simulink model "Disha_plant"  (R2026a)
settings: Solver=VariableStepAuto
settings Model: Creator=LENOVO  LastModifiedBy=LENOVO

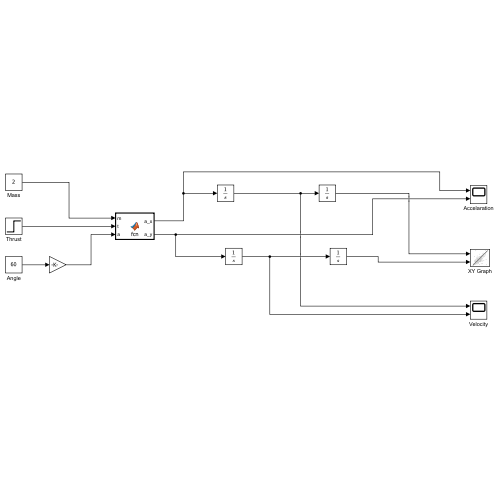
[thumbnail: Simulink's stored preview of the top-level diagram]
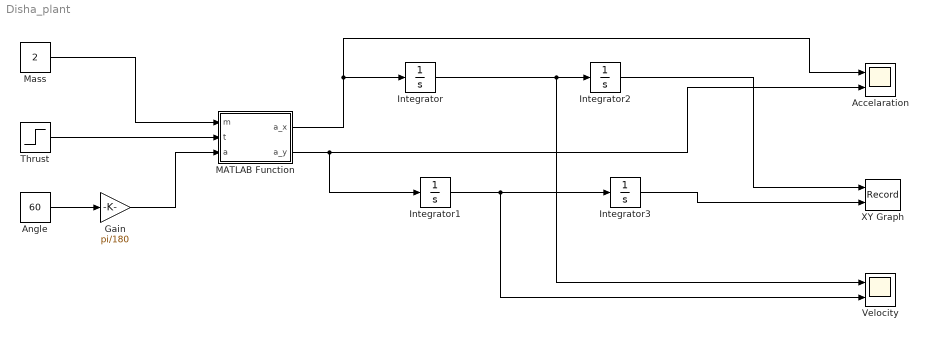
== system Disha_plant ==
  Accelaration : Scope  NumInputPorts=2
      settings: ActiveDisplayYMinimum=-0.0541265877365274  ActiveDisplayYMaximum=0.4871392896287467
  Angle : Constant  Value=60
  Gain : Gain  Gain=pi/180
  Integrator{,1..3} (4 alike) : Integrator
  MATLAB Function : MATLAB Function  TreatAsAtomicUnit=on
  Mass : Constant  Value=2
  Thrust : Step  SampleTime=0
  Velocity : Scope  NumInputPorts=2
      settings: ActiveDisplayYMinimum=-0.48713928962874653  ActiveDisplayYMaximum=4.38425360665872  DataLoggingVariableName=ScopeData2
  XY Graph : Record  NumPorts=2.0  FileSettingsInternal="{\"entries\":[{\"content\":{\"excelSettings\":{\"content\":{},\"type\":\"Streamout.ExcelSettings\"},\"parquetSettings\":{\"content\":{},\"type\":\"Streamout.ParquetSettings\"}},\"type\":\"Streamout.FileSettingStorage\",\"uuid\":\"\"}],\"packageUris\":[\"http:\\/\\/schema.mathworks.com\\/mf0\\/streamout_blocks\\/R2020a\"],\"version\":\"1.0\"}"  FrameSettings=[0, 0]  Layout=[1 1]  SignalsInternal="{\"entries\":[{\"content\":{\"signals\":[{\"content\":{\"blockPath\":[],\"dimensions\":[1],\"domain\":\"\",\"lineColor\":\"#a2142f\",\"plots\":[ 1 ],\"port\":1,\"sid\":[\"\"],\"signalID\":1,\"signalName\":\"Integrator2\"},\"type\":\"RecordBlkView.Signal\",\"uuid\":\"\"},{\"content\":{\"blockPath\":[],\"dimensions\":[1],\"domain\":\"\",\"lineColor\":\"#139fff\",\"plots\":[ 1 ],\"port\":2,\"sid\":[\"\"],\"signalID\":2,\"signalName\":\"Integrator3\"},\"type\":\"RecordBlkView.Signal\",\"uuid\":\"\"}]},\"type\":\"RecordBlkView.InputSignals\",\"uuid\":\"\"}],\"packageUris\":[\"http:\\/\\/schema.mathworks.com\\/mf0\\/streamout_blocks\\/R2020a\"],\"version\":\"1.0\"}"  VisualizationBindings="{\"xyplotplugin\":{\"info\":[{\"series\":[{\"bindingParametersList\":[{\"parameter\":\"X-Axis\",\"signalID\":1,\"signalName\":\"Integrator2\"},{\"parameter\":\"Y-Axis\",\"signalID\":2,\"signalName\":\"Integrator3\"}],\"seriesID\":0}],\"subplotID\":1}]}}"  CompatibilityTag=XY
  wires:
  Mass/1 -> MATLAB Function/1(m)
  Thrust/1 -> MATLAB Function/2(t)
  Angle/1 -> Gain/1
  Gain/1 -> MATLAB Function/3(a)
  MATLAB Function/2(a_y) -> Accelaration/2, Integrator1/1
  Integrator1/1 -> Velocity/2, Integrator3/1
  Integrator2/1 -> XY Graph/1
  Integrator3/1 -> XY Graph/2
  MATLAB Function/1(a_x) -> Accelaration/1, Integrator/1
  Integrator/1 -> Velocity/1, Integrator2/1

== matlab function Disha_plant/MATLAB Function ==
  data: m input; a_x output; t input; a input; a_y output
function [a_x, a_y] = fcn(m, t, a)
% Inputs:
%   m - mass (kg)
%   t - thrust (N)
%   a - thrust angle (rad, measured from vertical)
% Outputs:
%   a_x - horizontal acceleration (m/s^2)
%   a_y - vertical acceleration (m/s^2)

a_x = (t/m) * sin(a);
a_y = (t/m) * cos(a);

end
